simulink model "Traction_control"  (R2024b)
settings: Solver=VariableStepAuto  StartTime=0.0  StopTime=20  FixedStep=0.01  RelTol=1e-3
libraries: slpidlib x1
settings Model: Creator=Nikhil M  LastModifiedBy=Nikhil M
settings OptimizationCC: DefaultParameterBehavior=Inlined  EnhancedBackFolding=on  PassReuseOutputArgsAs=Individual arguments  ZeroExternalMemoryAtStartup=off  ZeroInternalMemoryAtStartup=off  OptimizeBlockOrder=speed  DifferentSizesBufferReuse=on  OptimizationCustomize=off  EfficientTunableParamExpr=on
settings DebuggingCC: ParameterTunabilityLossMsg=error
settings HardwareCC: ProdBitPerPointer=32  ProdBitPerSizeT=32  ProdBitPerPtrDiffT=32  ProdLargestAtomicInteger=Long  ProdLargestAtomicFloat=Double  ProdWordSize=32  ProdHWDeviceType=ARM Compatible->ARM Cortex-M
settings SFSimCC: MATLABDynamicMemAlloc=off
settings RTWCC: Description=Embedded Coder  SystemTargetFile=ert.tlc  TemplateMakefile=ert_default_tmf  TargetLang=C++
settings CodeAppCC: ForceParamTrailComments=on  IgnoreCustomStorageClasses=off  OperatorAnnotations=on  SimulinkDataObjDesc=on  SFDataObjDesc=on  InsertBlockDesc=on
settings ERTTargetCC: TargetLangStandard=C++11 (ISO)  GenerateSampleERTMain=on  CodeInterfacePackaging=C++ class  RootIOFormat=Structure reference  ERTCustomFileTemplate=example_file_process.tlc

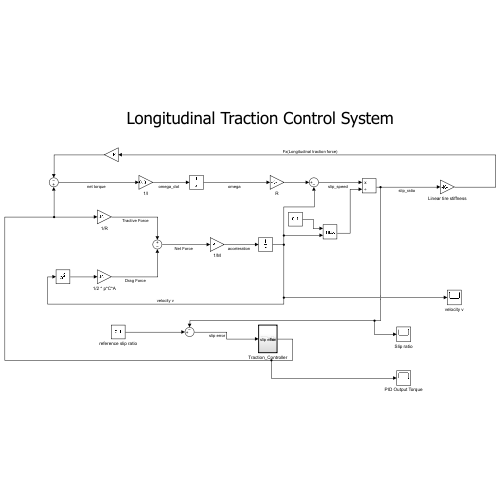
[thumbnail: Simulink's stored preview of the top-level diagram]
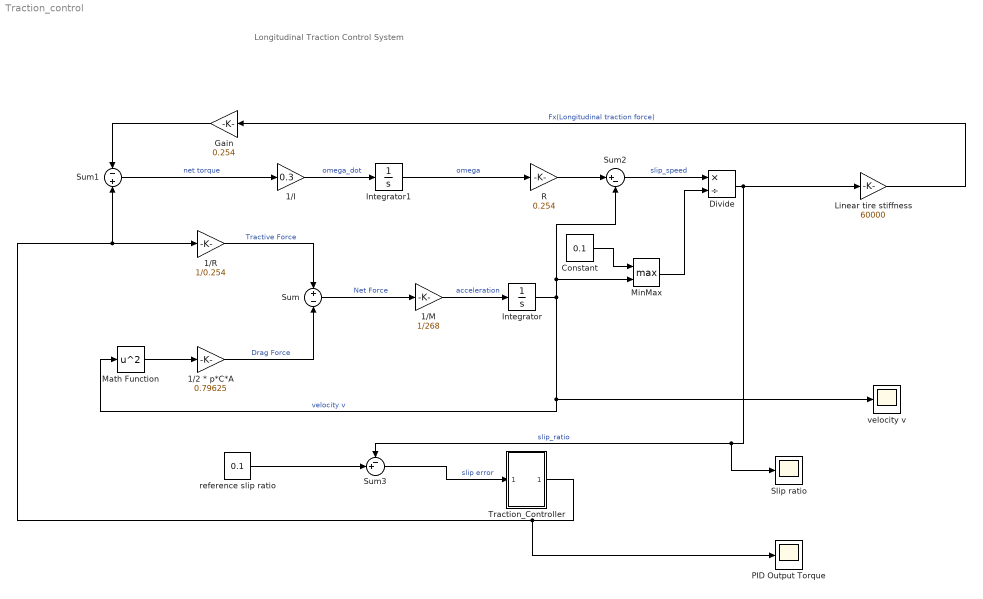
== system Traction_control ==
  note: Longitudinal Traction Control System
  1/2 * p*C*A : Gain  Gain=0.79625
  1/I : Gain  Gain=0.3
  1/M : Gain  Gain=1/268
  1/R : Gain  Gain=1/0.254
  Constant : Constant  Value=0.1
  Divide : Product  Inputs=*/
  Gain : Gain  Gain=0.254
  Integrator : Integrator
  Integrator1 : Integrator
  Linear tire stiffness : Gain  Gain=60000
  Math Function : Math  Operator=square
  MinMax : MinMax  Function=max  Inputs=2
  PID Output Torque : Scope
  R : Gain  Gain=0.254
  Slip ratio : Scope
  Sum : Sum  Inputs=+|-
  Sum1 : Sum  Inputs=-|+
  Sum2 : Sum  Inputs=|+-
  Sum3 : Sum  Inputs=-+|
  Traction_Controller : Subsystem  TreatAsAtomicUnit=on
  reference slip ratio : Constant  Value=0.1
  velocity v : Scope
  wires:
  Math Function/1 -> 1/2 * p*C*A/1
  1/2 * p*C*A/1 -> Sum/2  "Drag Force"
  1/R/1 -> Sum/1  "Tractive Force"
  Sum/1 -> 1/M/1  "Net Force"
  1/M/1 -> Integrator/1  "acceleration"
  Integrator/1 -> velocity v/1, Math Function/1, MinMax/2, Sum2/2  "velocity v"
  Sum1/1 -> 1/I/1  "net torque"
  1/I/1 -> Integrator1/1  "omega_dot"
  Integrator1/1 -> R/1  "omega"
  R/1 -> Sum2/1
  Constant/1 -> MinMax/1
  Sum2/1 -> Divide/1  "slip_speed"
  MinMax/1 -> Divide/2
  Divide/1 -> Slip ratio/1, Sum3/1, Linear tire stiffness/1  "slip_ratio"
  Gain/1 -> Sum1/1
  reference slip ratio/1 -> Sum3/2
  Linear tire stiffness/1 -> Gain/1  "Fx(Longitudinal traction force)"
  Traction_Controller/1(Tm) -> PID Output Torque/1, Sum1/2, 1/R/1
  Sum3/1 -> Traction_Controller/1(slip error)  "slip error"

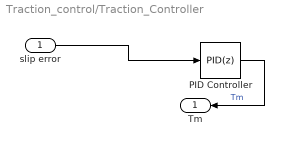
== system Traction_control/Traction_Controller ==
  slip error : Inport
  PID Controller : slpidlib/PID Controller  Controller=PID  Form=Parallel  TimeDomain=Discrete-time  UseExternalTs=off  SampleTime=0.01  IntegratorMethod=Forward Euler  FilterMethod=Forward Euler  ControllerParametersSource=internal  P=3000  I=1500  UseKiTs=off  D=0  UseExternalDerivativeSource=off  N=100  UseFilter=on  TunerSelectOption=Transfer Function Based (PID Tuner App)  InitialConditionSource=internal  InitialConditionForIntegrator=0  InitialConditionForFilter=0  DifferentiatorICPrevScaledInput=0  ExternalReset=none  TrackingMode=off  Kt=1  LimitOutput=on  SatLimitsSource=internal  UpperSaturationLimit=150  LowerSaturationLimit=0  LinearizeAsGain=on  AntiWindupMode=clamping  Kb=1  LimitIntegrator=off  UpperIntegratorSaturationLimit=inf  LowerIntegratorSaturationLimit=-inf  POutMin=[]  POutMax=[]  IOutMin=[]  IOutMax=[]  DOutMin=[]  DOutMax=[]  NOutMin=[]  NOutMax=[]  SumOutMin=[]  SumOutMax=[]  SaturationOutMin=[]  SaturationOutMax=[]  PParamMin=[]  PParamMax=[]  IParamMin=[]  IParamMax=[]  DParamMin=[]  DParamMax=[]  NParamMin=[]  NParamMax=[]  KbParamMin=[]  KbParamMax=[]  KtParamMin=[]  KtParamMax=[]  KbOutMin=[]  KbOutMax=[]  KtOutMin=[]  KtOutMax=[]  IntegratorOutMin=[]  IntegratorOutMax=[]  FilterOutMin=[]  FilterOutMax=[]  SumI1OutMin=[]  SumI1OutMax=[]  SumI2OutMin=[]  SumI2OutMax=[]  SumI3OutMin=[]  SumI3OutMax=[]  SumI4OutMin=[]  SumI4OutMax=[]  SumDOutMin=[]  SumDOutMax=[]  DifferentiatorOutMin=[]  DifferentiatorOutMax=[]  FilterDiffOutCoefMin=[]  FilterDiffOutCoefMax=[]  ReciprocalOutMin=[]  ReciprocalOutMax=[]  SumDenOutMin=[]  SumDenOutMax=[]  SumNumOutMin=[]  SumNumOutMax=[]  DivideOutMin=[]  DivideOutMax=[]  UdiffTsProdOutMin=[]  UdiffTsProdOutMax=[]  NTsProdOutMin=[]  NTsProdOutMax=[]  UintegralTsProdOutMin=[]  UintegralTsProdOutMax=[]  UngainTsProdOutMin=[]  UngainTsProdOutMax=[]  ClampingZeroOutDataTypeStr=Inherit: Inherit via back propagation  ClampingZeroOutMin=[]  ClampingZeroOutMax=[]  FilterDenConstantOutDataTypeStr=Inherit: Inherit via back propagation  FilterDenConstantOutMin=[]  FilterDenConstantOutMax=[]  PCopyOutDataTypeStr=Inherit: Inherit via back propagation  PCopyOutMin=[]  PCopyOutMax=[]  NCopyOutDataTypeStr=Inherit: Inherit via back propagation  NCopyOutMin=[]  NCopyOutMax=[]  IntegratorContinuousStateAttributes=''  IntegratorStateMustResolveToSignalObject=off  IntegratorRTWStateStorageClass=Auto  FilterContinuousStateAttributes=''  FilterStateMustResolveToSignalObject=off  FilterRTWStateStorageClass=Auto  ParallelPVariant=InternalParameters  IdealPVariant=Disabled  IVariant=InternalParameters  DVariant=InternalParameters  IntegratorVariant=Discrete  SatVariant=Enabled  AWVariant=DiscClampingParallel  PCopyVariant=Disabled  TRVariant=Disabled  FdbkBlocksVariant=Forward  IdealPFdbkVariant=Disabled  SatFdbkVariant=Disabled  DerivativeFilterVariant=ForwardEulerFilter  NVariant=InternalParameters  NCopyVariant=Disabled  FilterICVariant=InternalICsFilter  IntegratorICVariant=InternalICs  ExternalResetVariant=Disabled  TRSumVariant=Passthrough  SumFdbkVariant=Disabled  SumVariant=Sum_PID  TsampFilterVariant=InternalTs  TsampNgainVariant=Passthrough  TsampIntegralVariant=Disabled_SignalSpec  ExternalSaturationOutDataTypeStr=Inherit: Same as second input  DerivativeSourceVariant=ErrorSignal  PreIntVariant=InternalPreInt
  Tm : Outport
  wires:
  PID Controller/1 -> Tm/1  "Tm"
  slip error/1 -> PID Controller/1
